simulink model "simulinkModel"  (R2024b)
settings: Solver=VariableStepAuto  StartTime=0.0  StopTime=1  RelTol=1e-3
libraries: spsDiodeLib x10, spsSeriesRLCBranchLib x6, spsVoltageMeasurementLib x6, spsCurrentMeasurementLib x4, spsACVoltageSourceLib x2, spsMosfetLib x2, fuzblock x1, eeGeneralControl x1, spsPLLLib x1, sps_lib x1
settings Model: Creator=Sandeep Athreya  LastModifiedBy=Sandeep Athreya

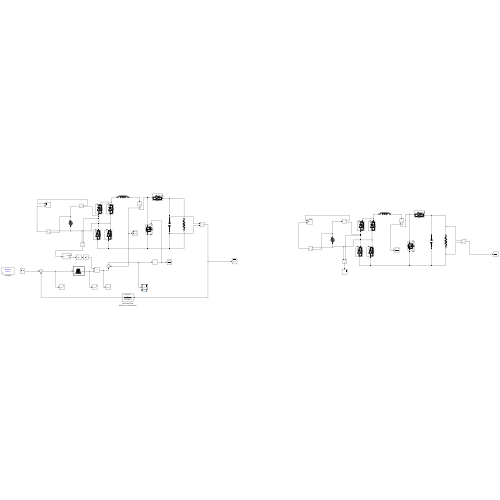
[thumbnail: Simulink's stored preview of the top-level diagram]
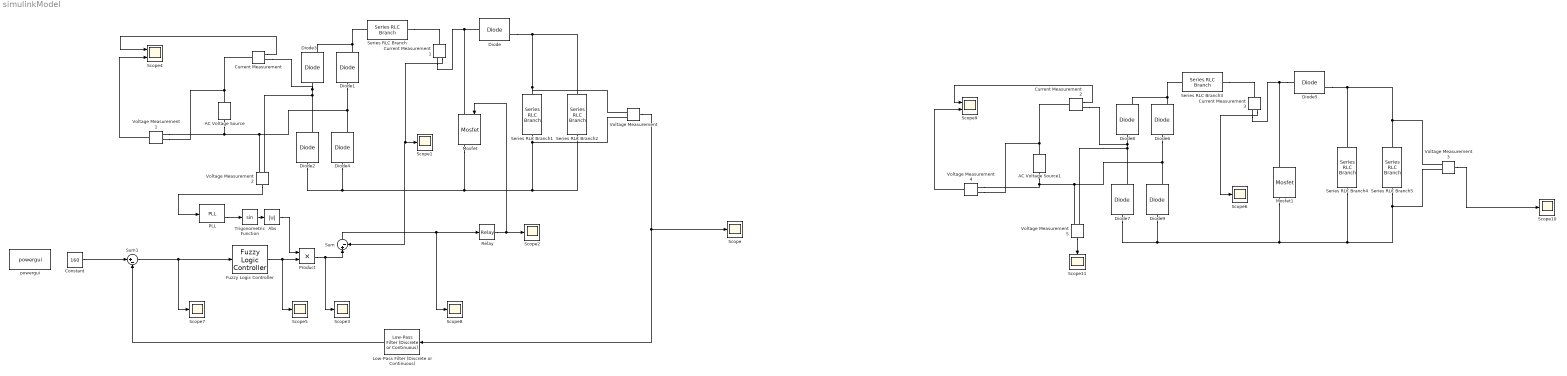
== system simulinkModel ==
  AC Voltage Source : spsACVoltageSourceLib/AC Voltage Source  Amplitude=150  Phase=0  Frequency=50  SampleTime=0  Measurements=None  BusType=swing  Pref=10e3  Qref=0  Qmin=-inf  Qmax=+inf
  AC Voltage Source1 : spsACVoltageSourceLib/AC Voltage Source  Amplitude=150  Phase=0  Frequency=50  SampleTime=0  Measurements=None  BusType=swing  Pref=10e3  Qref=0  Qmin=-inf  Qmax=+inf
  Abs : Abs  SaturateOnIntegerOverflow=off
  Constant : Constant  Value=160
  Current Measurement{,1..3} (4 alike) : spsCurrentMeasurementLib/Current Measurement  PhasorSimulation=off  OutputType=Complex  PSBequivalent=0
  Diode : spsDiodeLib/Diode  Ron=0.001  Lon=0  Vf=0.8  IC=0  UseSnubber=0  Rs=1e5  Cs=1e-9  Measurements=on
  Diode{1..4,6..9} (8 alike) : spsDiodeLib/Diode  Ron=0.001  Lon=0  Vf=0.8  IC=0  UseSnubber=0  Rs=500  Cs=250e-9  Measurements=on
  Diode5 : spsDiodeLib/Diode  Ron=0.001  Lon=0  Vf=0.8  IC=0  UseSnubber=0  Rs=1e5  Cs=1e-9  Measurements=on
  Fuzzy Logic Controller : fuzblock/Fuzzy Logic  Controller  FIS=fis  OutputSampleNumber=101  DataType=double  FuzzifiedInputs=off  RuleFiringStrengths=off  RuleOutputs=off  AggregatedOutputs=off  SimulateUsing=Interpreted execution  OutOfRangeInputValueMessage=warning  NoRuleFiredMessage=warning  EmptyOutputFuzzySetMessage=warning
  Low-Pass Filter (Discrete or Continuous) : eeGeneralControl/Low-Pass Filter (Discrete or Continuous)  K=1  T=0.0159  B=inf  A=-inf  init_option=Inherited from block input  x0=0  Ts=0.05
  Mosfet : spsMosfetLib/Mosfet  Ron=0.1  Lon=0  Rd=0.01  Vfd=0  IC=0  Rs=1e5  Cs=1e-9  Measurements=on
  Mosfet1 : spsMosfetLib/Mosfet  Ron=0.1  Lon=0  Rd=0.01  Vfd=0  IC=0  Rs=1e5  Cs=1e-9  Measurements=on
  PLL : spsPLLLib/PLL  Fmin=15  Par_Init=[0, 50]  ParK=[180, 3200, 1]  TcD=1e-4  MaxRateChangeFreq=12  FilterCutOffFreq=25  Ts=0  AGC=on
      settings: LibrarySourceBlock=sps_lib/Control/PLL
  Product : Product
  Relay : Relay  OnSwitchValue=0.1  OffSwitchValue=-0.1
  Scope{,1..3,5..8,10..11} (10 alike) : Scope
  Scope4 : Scope  NumInputPorts=2
  Scope9 : Scope  NumInputPorts=2
  Series RLC Branch : spsSeriesRLCBranchLib/Series RLC Branch  LConnTagsString=__new0  RConnTagsString=__new0  BranchType=L  Resistance=1  Inductance=22.5e-3  SetiL0=off  InitialCurrent=0  Capacitance=1e-6  Setx0=off  InitialVoltage=0  Measurements=None
  Series RLC Branch1 : spsSeriesRLCBranchLib/Series RLC Branch  LConnTagsString=__new0  RConnTagsString=__new0  BranchType=C  Resistance=1  Inductance=1e-3  SetiL0=off  InitialCurrent=0  Capacitance=940e-6  Setx0=off  InitialVoltage=0  Measurements=None
  Series RLC Branch2 : spsSeriesRLCBranchLib/Series RLC Branch  LConnTagsString=__new0  RConnTagsString=__new0  BranchType=R  Resistance=212  Inductance=1e-3  SetiL0=off  InitialCurrent=0  Capacitance=1e-6  Setx0=off  InitialVoltage=0  Measurements=None
  Series RLC Branch3 : spsSeriesRLCBranchLib/Series RLC Branch  LConnTagsString=__new0  RConnTagsString=__new0  BranchType=L  Resistance=1  Inductance=22.5e-3  SetiL0=off  InitialCurrent=0  Capacitance=1e-6  Setx0=off  InitialVoltage=0  Measurements=None
  Series RLC Branch4 : spsSeriesRLCBranchLib/Series RLC Branch  LConnTagsString=__new0  RConnTagsString=__new0  BranchType=C  Resistance=1  Inductance=1e-3  SetiL0=off  InitialCurrent=0  Capacitance=940e-6  Setx0=off  InitialVoltage=0  Measurements=None
  Series RLC Branch5 : spsSeriesRLCBranchLib/Series RLC Branch  LConnTagsString=__new0  RConnTagsString=__new0  BranchType=R  Resistance=212  Inductance=1e-3  SetiL0=off  InitialCurrent=0  Capacitance=1e-6  Setx0=off  InitialVoltage=0  Measurements=None
  Sum : Sum  Inputs=|+-
  Sum1 : Sum  Inputs=|+-
  Trigonometric Function : Trigonometry
  Voltage Measurement{,1..5} (6 alike) : spsVoltageMeasurementLib/Voltage Measurement  PhasorSimulation=off  OutputType=Complex  PSBequivalent=0
  powergui : sps_lib/powergui  Priority=1  SimulationMode=Discrete  SampleTime=1e-6  frequency=60  Iterations=50  frequencyindice=50  Pbase=100e6  ErrMax=1e-4  UnitsV=kV  UnitsW=MW  buscounter=0  FunctionMessages=off  echomessages=off  EnableUseOfTLC=off  CurrentSourceSwitches=off  DisableSnubberDevices=off  DisableRonSwitches=off  DisableVfSwitches=off  DisplayEquations=off  AutomaticDiscreteSolvers=off  SolverType=Tustin/Backward Euler (TBE)  Interpol=off  ExternalGateDelay=off  methode=off  Ts=100  x0status=blocks  SPID=on  SwTol=0  HookPort=off  NonlinearTolerance=1e-4  nMaxIteration=100  ContinueOnMaxIteration=off  RestoreLinks=warning  ResistiveCurrentMeasurement=off  Frange=[0:2:500]  Ylog=off  Xlog=on  ShowGrid=off  save=off  variable=ZData  structure=0  ZoomFFT=off  StartTime=0.0  cycles=1  DisplayStyle=1  fundamental=60  FreqAxis=off  MaxFrequency=1000  frequencyindicesteady=1  RmsSteady=1  display=off
  wires:
  Current Measurement/1 -> Scope4/1
  Sum1/1 -> Scope7/1, Fuzzy Logic Controller/1
  Constant/1 -> Sum1/1
  Voltage Measurement1/1 -> Scope4/2
  Voltage Measurement/1 -> Low-Pass Filter (Discrete or Continuous)/1, Scope/1
  Low-Pass Filter (Discrete or Continuous)/1 -> Sum1/2
  Fuzzy Logic Controller/1 -> Scope5/1, Product/2
  Voltage Measurement2/1 -> PLL/1
  Product/1 -> Scope3/1, Sum/1
  Sum/1 -> Scope8/1, Relay/1
  Relay/1 -> Mosfet/1, Scope2/1
  Current Measurement1/1 -> Sum/2, Scope1/1
  PLL/2 -> Trigonometric Function/1
  Trigonometric Function/1 -> Abs/1
  Abs/1 -> Product/1
  Voltage Measurement4/1 -> Scope9/2
  Current Measurement3/1 -> Scope6/1
  Current Measurement2/1 -> Scope9/1
  Voltage Measurement3/1 -> Scope10/1
  Voltage Measurement5/1 -> Scope11/1
  connections:
  Series RLC Branch1/RConn1 -- Series RLC Branch2/RConn1 -- Diode4/LConn1 -- Diode2/LConn1 -- Mosfet/RConn1 -- Voltage Measurement/LConn2
  Mosfet/LConn1 -- Current Measurement1/RConn1 -- Diode/LConn1
  Diode2/RConn1 -- Current Measurement/RConn1 -- Diode3/LConn1 -- Voltage Measurement2/LConn1
  Series RLC Branch2/LConn1 -- Voltage Measurement/LConn1 -- Series RLC Branch1/LConn1 -- Diode/RConn1
  Diode1/LConn1 -- AC Voltage Source/LConn1 -- Voltage Measurement1/LConn2 -- Voltage Measurement2/LConn2 -- Diode4/RConn1
  Diode3/RConn1 -- Series RLC Branch/LConn1 -- Diode1/RConn1
  Current Measurement/LConn1 -- Voltage Measurement1/LConn1 -- AC Voltage Source/RConn1
  Series RLC Branch/RConn1 -- Current Measurement1/LConn1
  Diode6/RConn1 -- Series RLC Branch3/LConn1 -- Diode8/RConn1
  Voltage Measurement5/LConn2 -- Diode6/LConn1 -- Diode9/RConn1 -- AC Voltage Source1/LConn1 -- Voltage Measurement4/LConn2
  Mosfet1/RConn1 -- Diode9/LConn1 -- Diode7/LConn1 -- Series RLC Branch4/RConn1 -- Series RLC Branch5/RConn1 -- Voltage Measurement3/LConn2
  Diode5/LConn1 -- Mosfet1/LConn1 -- Current Measurement3/RConn1
  Series RLC Branch5/LConn1 -- Series RLC Branch4/LConn1 -- Diode5/RConn1 -- Voltage Measurement3/LConn1
  Current Measurement2/LConn1 -- Voltage Measurement4/LConn1 -- AC Voltage Source1/RConn1
  Diode7/RConn1 -- Voltage Measurement5/LConn1 -- Current Measurement2/RConn1 -- Diode8/LConn1
  Series RLC Branch3/RConn1 -- Current Measurement3/LConn1
